simulink model "Modelo_Lazo_Cerrado_Discretizado"  (R2026b)
settings: Solver=VariableStepAuto
values from neighbouring files (symbols this model uses):
  alpha_Cu = 3.9e-3    (= 0.0039)    [coeficientes.m]
  b_eq = b_m + b_l/(r^2)    (= 2.19444444444e-05)    [coeficientes.m]
  C_ts = 0.818    [coeficientes.m]
  g = 9.80665    [coeficientes.m]
  init_I0 = 0    [coeficientes.m]
  init_Id = 0    [coeficientes.m]
  init_Iq = 0    [coeficientes.m]
  init_theta = 0    [coeficientes.m]
  init_Ts = 20    [coeficientes.m]
  init_w = 0    [coeficientes.m]
  J_eq = J_m + J_l/(r^2)    (= 4.58263888889e-05)    [coeficientes.m]
  K_et = 2*p_obs    (= 6400)    [coeficientes.m]
  K_ew = p_obs^2    (= 10240000)    [coeficientes.m]
  k_l = k_l_min + m_l*l_l    (= 1)    [coeficientes.m]
  Kd_mov = wn_mov * (2*zeta_mov + 1) * J_eq    (= 0.0916527777778)    [coeficientes.m]
  Ki_mov = wn_mov^3 * J_eq    (= 23463.1111111)    [coeficientes.m]
  Kp_mov = wn_mov^2 * (2*zeta_mov + 1) * J_eq    (= 73.3222222222)    [coeficientes.m]
  L_d = 6.6e-3    (= 0.0066)    [coeficientes.m]
  L_ls = 0.8e-3    (= 0.0008)    [coeficientes.m]
  L_q = 5.8e-3    (= 0.0058)    [coeficientes.m]
  lambda = 0.016    [coeficientes.m]
  Pp = 3    [coeficientes.m]
  r = 120.0    (= 120)    [coeficientes.m]
  R0 = abs(p)*L_ls    [coeficientes.m]
  R_sREF = 1.02    [coeficientes.m]
  R_tsamb = 146.7    [coeficientes.m]
  Rd = abs(p)*L_d    [coeficientes.m]
  Rq = abs(p)*L_q    [coeficientes.m]
  sat_V = sqrt(2/3)*V_slMAX    [coeficientes.m]
  T_sREF = 20    [coeficientes.m]
  Ts = 1e-5    (= 1e-05)    [coeficientes.m]
libraries: eeTransforms x4, eeGeneralControl x3
settings Model: Creator=fedeb  LastModifiedBy=fedeb

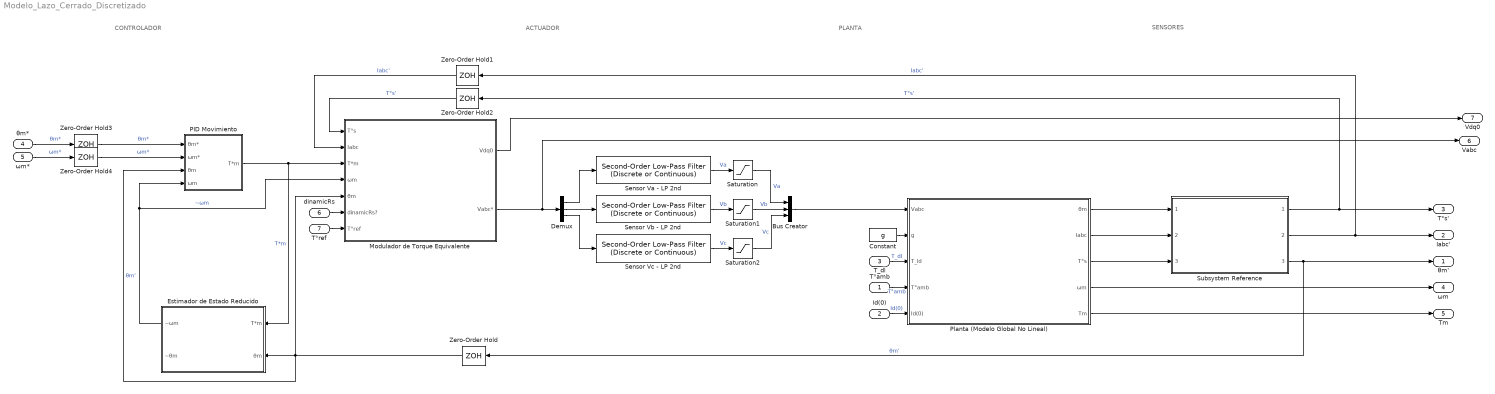
== system Modelo_Lazo_Cerrado_Discretizado ==
  note: PLANTA
  note: SENSORES
  note: CONTROLADOR
  note: ACTUADOR
  T°amb : Inport
  Id(0) : Inport  Port=2
  T_dl : Inport  Port=3
  θm* : Inport  Port=4
  ωm* : Inport  Port=5
  dinamicRs : Inport  Port=6
  T°ref : Inport  Port=7
  Bus Creator : BusCreator  Inputs=3
  Constant : Constant  Value=g
  Demux : Demux  Outputs=3
  Estimador de Estado Reducido : Subsystem
  Modulador de Torque Equivalente : Subsystem
      settings: PortSchema="{\"entries\":[{\"content\":{\"sides\":[{\"content\":{\"connectorIds\":[\"In1\",\"In3\",\"In5\",\"In2\",\"In4\",\"In6\",\"In7\"]},\"type\":\"ConnectorPlacement.EquallySpacedRectSide\",\"uuid\":\"ea9ad4ab-f607-4d37-9442-85f6cfda2486\"},{\"content\":{\"connectorIds\":[\"Out2\",\"Out1\"],\"side\":\"RIGHT\"},\"type\":\"ConnectorPlacement.EquallySpacedRectSide\",\"uuid\":\"696b5fe5-1f6c-4fc9-932e-86b56d49996f\"},{\"content\":{\"side\":\"TOP\"},\"type\":\"ConnectorPlacement.EquallySpacedRectSide\",\"uuid\":\"45e3ac4c-5a2f-4a79-9454-e497b07295c7\"}]},\"type\":\"ConnectorPlacement.EquallySpacedConnector\",\"uuid\":\"ad401c21-3c60-4ab4-96eb-f449fc93609a\"}],\"packageUris\":[\"http://schema.mathworks.com/mf0/Connector/R2020b\"],\"version\":\"1.0\"}"
  PID Movimiento : Subsystem
      settings: PortSchema="{\"entries\":[{\"content\":{\"sides\":[{\"content\":{\"connectorIds\":[\"In3\",\"In4\",\"In2\",\"In1\"]},\"type\":\"ConnectorPlacement.EquallySpacedRectSide\",\"uuid\":\"99b9ec4b-f651-40ed-8a16-085c2c4ac88d\"},{\"content\":{\"connectorIds\":[\"Out1\"],\"side\":\"RIGHT\"},\"type\":\"ConnectorPlacement.EquallySpacedRectSide\",\"uuid\":\"009a9369-fd86-4ac2-a423-7c7f1491457b\"},{\"content\":{\"side\":\"TOP\"},\"type\":\"ConnectorPlacement.EquallySpacedRectSide\",\"uuid\":\"0bc889a5-9100-482e-a11a-4c36993d76f7\"}]},\"type\":\"ConnectorPlacement.EquallySpacedConnector\",\"uuid\":\"de270b8a-8a15-46e7-87f3-10db7988a399\"}],\"packageUris\":[\"http://schema.mathworks.com/mf0/Connector/R2020b\"],\"version\":\"1.0\"}"
  Planta (Modelo Global No Lineal) : Subsystem
      settings: PortSchema="{\"entries\":[{\"content\":{\"sides\":[{\"content\":{\"connectorIds\":[\"In1\",\"In3\",\"In2\",\"In4\",\"In5\"]},\"type\":\"ConnectorPlacement.EquallySpacedRectSide\",\"uuid\":\"3481abf0-b0cb-49f6-b93f-5a31fbfa4119\"},{\"content\":{\"connectorIds\":[\"Out1\",\"Out2\",\"Out3\",\"Out4\",\"Out5\"],\"side\":\"RIGHT\"},\"type\":\"ConnectorPlacement.EquallySpacedRectSide\",\"uuid\":\"81dbc61e-d5f3-4edc-bc73-ec3d6160a008\"},{\"content\":{\"side\":\"TOP\"},\"type\":\"ConnectorPlacement.EquallySpacedRectSide\",\"uuid\":\"48e37594-92fb-4835-b4aa-9211b8b6a309\"}]},\"type\":\"ConnectorPlacement.EquallySpacedConnector\",\"uuid\":\"6c32b8e1-5803-41f4-af4e-ba3a494349ba\"}],\"packageUris\":[\"http://schema.mathworks.com/mf0/Connector/R2020b\"],\"version\":\"1.0\"}"
  Saturation : Saturate  UpperLimit=sat_V  LowerLimit=-sat_V
  Saturation1 : Saturate  UpperLimit=sat_V  LowerLimit=-sat_V
  Saturation2 : Saturate  UpperLimit=sat_V  LowerLimit=-sat_V
  Sensor Va - LP 2nd : eeGeneralControl/Second-Order Low-Pass Filter (Discrete or Continuous)  A1=A1_V  A2=A2_V  init_option=Inherited from block input  x0=0  Ts=0
      settings: LibrarySourceBlock=|
      | ee_sl_lib/General Control/Second-Order
      | Low-Pass Filter
      | (Discrete or Continuous)
  Sensor Vb - LP 2nd : eeGeneralControl/Second-Order Low-Pass Filter (Discrete or Continuous)  A1=A1_V  A2=A2_V  init_option=Inherited from block input  x0=0  Ts=0
      settings: LibrarySourceBlock=|
      | ee_sl_lib/General Control/Second-Order
      | Low-Pass Filter
      | (Discrete or Continuous)
  Sensor Vc - LP 2nd : eeGeneralControl/Second-Order Low-Pass Filter (Discrete or Continuous)  A1=A1_V  A2=A2_V  init_option=Inherited from block input  x0=0  Ts=0
      settings: LibrarySourceBlock=|
      | ee_sl_lib/General Control/Second-Order
      | Low-Pass Filter
      | (Discrete or Continuous)
  Subsystem Reference : Subsystem  ReferencedSubsystem=Sensores_Reales
  Zero-Order Hold{,1..4} (5 alike) : ZeroOrderHold  SampleTime=Ts
  θm' : Outport
  Iabc' : Outport  Port=2  OutDataTypeStr=Bus: Iabc
  T°s' : Outport  Port=3
  ωm : Outport  Port=4
  Tm : Outport  Port=5
  Vabc : Outport  Port=6  OutDataTypeStr=Bus: Vabc
  Vdq0 : Outport  Port=7  OutDataTypeStr=Bus: Vdq0
  wires:
  ωm*/1 -> Zero-Order Hold4/1  "ωm*"
  dinamicRs/1 -> Modulador de Torque Equivalente/6(dinamicRs?)
  Modulador de Torque Equivalente/2(Vdq0) -> Vdq0/1
  Planta (Modelo Global No Lineal)/5(Tm) -> Tm/1
  θm*/1 -> Zero-Order Hold3/1  "θm*"
  T_dl/1 -> Planta (Modelo Global No Lineal)/2(T_ld)  "T_dl"
  Planta (Modelo Global No Lineal)/4(ωm) -> ωm/1
  T°ref/1 -> Modulador de Torque Equivalente/7(T°ref)
  Id(0)/1 -> Planta (Modelo Global No Lineal)/5(Id(0))  "Id(0)"
  T°amb/1 -> Planta (Modelo Global No Lineal)/4(T°amb)  "T°amb"
  Subsystem Reference/2 -> Iabc'/1, Zero-Order Hold1/1  "Iabc'"
  Constant/1 -> Planta (Modelo Global No Lineal)/3(g)
  Subsystem Reference/1 -> T°s'/1, Zero-Order Hold2/1  "T°s'"
  Estimador de Estado Reducido/1(~ωm) -> Modulador de Torque Equivalente/2(ωm), PID Movimiento/1(ωm)  "~ωm"
  PID Movimiento/1(T*m) -> Modulador de Torque Equivalente/5(T*m), Estimador de Estado Reducido/1(T*m)  "T*m"
  Planta (Modelo Global No Lineal)/2(Iabc) -> Subsystem Reference/2
  Planta (Modelo Global No Lineal)/3(T°s) -> Subsystem Reference/3
  Planta (Modelo Global No Lineal)/1(θm) -> Subsystem Reference/1
  Subsystem Reference/3 -> θm'/1, Zero-Order Hold/1  "θm'"
  Sensor Va - LP 2nd/1 -> Saturation/1  "Va"
  Bus Creator/1 -> Planta (Modelo Global No Lineal)/1(Vabc)
  Saturation/1 -> Bus Creator/1  "Va"
  Sensor Vb - LP 2nd/1 -> Saturation1/1  "Vb"
  Saturation2/1 -> Bus Creator/3  "Vc"
  Demux/3 -> Sensor Vc - LP 2nd/1
  Modulador de Torque Equivalente/1(Vabc*) -> Demux/1, Vabc/1
  Demux/2 -> Sensor Vb - LP 2nd/1
  Demux/1 -> Sensor Va - LP 2nd/1
  Sensor Vc - LP 2nd/1 -> Saturation2/1  "Vc"
  Saturation1/1 -> Bus Creator/2  "Vb"
  Zero-Order Hold/1 -> Estimador de Estado Reducido/2(θm), PID Movimiento/2(θm), Modulador de Torque Equivalente/4(θm)  "θm'"
  Zero-Order Hold1/1 -> Modulador de Torque Equivalente/3(Iabc)  "Iabc'"
  Zero-Order Hold2/1 -> Modulador de Torque Equivalente/1(T°s)  "T°s'"
  Zero-Order Hold3/1 -> PID Movimiento/3(θm*)  "θm*"
  Zero-Order Hold4/1 -> PID Movimiento/4(ωm*)  "ωm*"

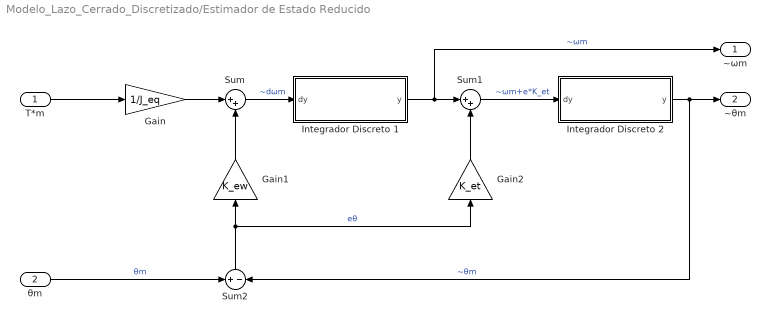
== system Modelo_Lazo_Cerrado_Discretizado/Estimador de Estado Reducido ==
  T*m : Inport
  θm : Inport  Port=2
  Gain : Gain  Gain=1/J_eq
  Gain1 : Gain  Gain=K_ew
  Gain2 : Gain  Gain=K_et
  Integrador Discreto 1 : Subsystem
  Integrador Discreto 2 : Subsystem
  Sum : Sum  Inputs=|++
  Sum1 : Sum  Inputs=|++
  Sum2 : Sum  Inputs=+-
  ~ωm : Outport
  ~θm : Outport  Port=2
  wires:
  T*m/1 -> Gain/1
  Gain/1 -> Sum/1
  Sum/1 -> Integrador Discreto 1/1(dy)  "~dωm"
  Sum1/1 -> Integrador Discreto 2/1(dy)  "~ωm+e*K_et"
  Integrador Discreto 1/1(y) -> ~ωm/1, Sum1/1  "~ωm"
  Gain1/1 -> Sum/2
  Gain2/1 -> Sum1/2
  Sum2/1 -> Gain1/1, Gain2/1  "eθ"
  θm/1 -> Sum2/1  "θm"
  Integrador Discreto 2/1(y) -> Sum2/2, ~θm/1  "~θm"

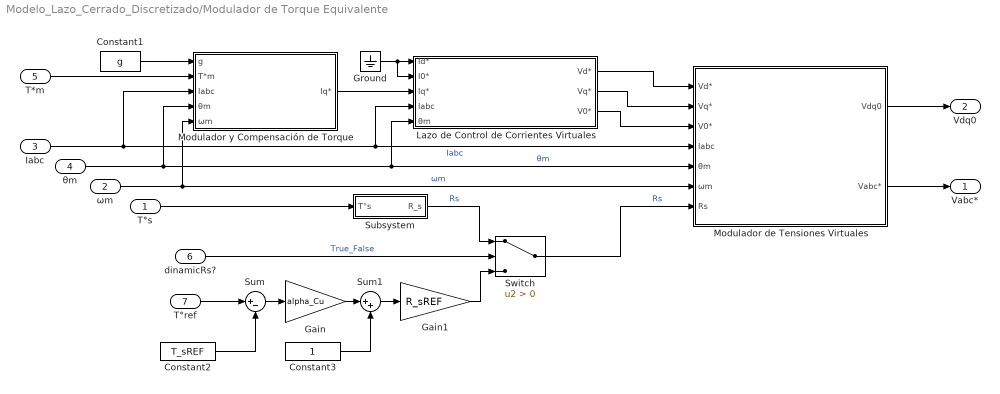
== system Modelo_Lazo_Cerrado_Discretizado/Modulador de Torque Equivalente ==
  T°s : Inport
  ωm : Inport  Port=2
  Iabc : Inport  Port=3
  θm : Inport  Port=4
  T*m : Inport  Port=5
  dinamicRs? : Inport  Port=6
  T°ref : Inport  Port=7
  Constant1 : Constant  Value=g
  Constant2 : Constant  Value=T_sREF
  Constant3 : Constant
  Gain : Gain  Gain=alpha_Cu
  Gain1 : Gain  Gain=R_sREF
  Ground : Ground
  Lazo de Control de Corrientes Virtuales : Subsystem
      settings: PortSchema="{\"entries\":[{\"content\":{\"sides\":[{\"content\":{\"connectorIds\":[\"In2\",\"In3\",\"In1\",\"In4\",\"In5\"]},\"type\":\"ConnectorPlacement.EquallySpacedRectSide\",\"uuid\":\"7378df2b-1b9c-42cd-9ef6-9bfa4de31228\"},{\"content\":{\"connectorIds\":[\"Out2\",\"Out1\",\"Out3\"],\"side\":\"RIGHT\"},\"type\":\"ConnectorPlacement.EquallySpacedRectSide\",\"uuid\":\"75ac4e09-b611-4ee2-aa1e-16791f3f98b8\"},{\"content\":{\"side\":\"TOP\"},\"type\":\"ConnectorPlacement.EquallySpacedRectSide\",\"uuid\":\"c32b7829-5b6a-417b-8aae-eaa4caf59bef\"}]},\"type\":\"ConnectorPlacement.EquallySpacedConnector\",\"uuid\":\"1d84f5ff-db01-492a-bfe1-22065b3eebb0\"}],\"packageUris\":[\"http://schema.mathworks.com/mf0/Connector/R2020b\"],\"version\":\"1.0\"}"
  Modulador de Tensiones Virtuales : Subsystem
      settings: PortSchema="{\"entries\":[{\"content\":{\"sides\":[{\"content\":{\"connectorIds\":[\"In2\",\"In1\",\"In3\",\"In6\",\"In7\",\"In5\",\"In4\"]},\"type\":\"ConnectorPlacement.EquallySpacedRectSide\",\"uuid\":\"561a625a-719f-47d4-85d3-a88e423068dd\"},{\"content\":{\"connectorIds\":[\"Out2\",\"Out1\"],\"side\":\"RIGHT\"},\"type\":\"ConnectorPlacement.EquallySpacedRectSide\",\"uuid\":\"c1cdd74a-6c1d-470e-a6ac-8d72e83b5cc5\"},{\"content\":{\"side\":\"TOP\"},\"type\":\"ConnectorPlacement.EquallySpacedRectSide\",\"uuid\":\"c5935c6f-534c-46b9-aa64-6d6dabbbb210\"}]},\"type\":\"ConnectorPlacement.EquallySpacedConnector\",\"uuid\":\"b0debde9-6e18-4e06-b0c4-28c9c51e472d\"}],\"packageUris\":[\"http://schema.mathworks.com/mf0/Connector/R2020b\"],\"version\":\"1.0\"}"
  Modulador y Compensación de Torque : Subsystem
      settings: PortSchema="{\"entries\":[{\"content\":{\"sides\":[{\"content\":{\"connectorIds\":[\"In5\",\"In1\",\"In2\",\"In3\",\"In4\"]},\"type\":\"ConnectorPlacement.EquallySpacedRectSide\",\"uuid\":\"ea9ad4ab-f607-4d37-9442-85f6cfda2486\"},{\"content\":{\"connectorIds\":[\"Out1\"],\"side\":\"RIGHT\"},\"type\":\"ConnectorPlacement.EquallySpacedRectSide\",\"uuid\":\"696b5fe5-1f6c-4fc9-932e-86b56d49996f\"},{\"content\":{\"side\":\"TOP\"},\"type\":\"ConnectorPlacement.EquallySpacedRectSide\",\"uuid\":\"45e3ac4c-5a2f-4a79-9454-e497b07295c7\"}]},\"type\":\"ConnectorPlacement.EquallySpacedConnector\",\"uuid\":\"ad401c21-3c60-4ab4-96eb-f449fc93609a\"}],\"packageUris\":[\"http://schema.mathworks.com/mf0/Connector/R2020b\"],\"version\":\"1.0\"}"
  Subsystem : Subsystem
  Sum : Sum  Inputs=|+-
  Sum1 : Sum  Inputs=|++
  Switch : Switch  Criteria=u2 > Threshold  SaturateOnIntegerOverflow=off  InputSameDT=off
  Vabc* : Outport
  Vdq0 : Outport  Port=2
  wires:
  Lazo de Control de Corrientes Virtuales/1(Vq*) -> Modulador de Tensiones Virtuales/1(Vq*)
  Lazo de Control de Corrientes Virtuales/2(Vd*) -> Modulador de Tensiones Virtuales/2(Vd*)
  Lazo de Control de Corrientes Virtuales/3(V0*) -> Modulador de Tensiones Virtuales/3(V0*)
  Modulador y Compensación de Torque/1(Iq*) -> Lazo de Control de Corrientes Virtuales/1(Iq*)
  T*m/1 -> Modulador y Compensación de Torque/1(T*m)
  θm/1 -> Modulador de Tensiones Virtuales/7(θm), Lazo de Control de Corrientes Virtuales/5(θm), Modulador y Compensación de Torque/3(θm)  "θm"
  ωm/1 -> Modulador de Tensiones Virtuales/5(ωm), Modulador y Compensación de Torque/4(ωm)  "ωm"
  Modulador de Tensiones Virtuales/1(Vabc*) -> Vabc*/1
  Ground/1 -> Lazo de Control de Corrientes Virtuales/2(Id*), Lazo de Control de Corrientes Virtuales/3(I0*)
  Iabc/1 -> Modulador de Tensiones Virtuales/6(Iabc), Lazo de Control de Corrientes Virtuales/4(Iabc), Modulador y Compensación de Torque/2(Iabc)  "Iabc"
  T°s/1 -> Subsystem/1(T°s)
  Subsystem/1(R_s) -> Switch/1  "Rs"
  dinamicRs?/1 -> Switch/2  "True_False"
  Switch/1 -> Modulador de Tensiones Virtuales/4(Rs)  "Rs"
  Gain1/1 -> Switch/3
  Modulador de Tensiones Virtuales/2(Vdq0) -> Vdq0/1
  Constant1/1 -> Modulador y Compensación de Torque/5(g)
  T°ref/1 -> Sum/1
  Constant2/1 -> Sum/2
  Sum/1 -> Gain/1
  Gain/1 -> Sum1/1
  Constant3/1 -> Sum1/2
  Sum1/1 -> Gain1/1

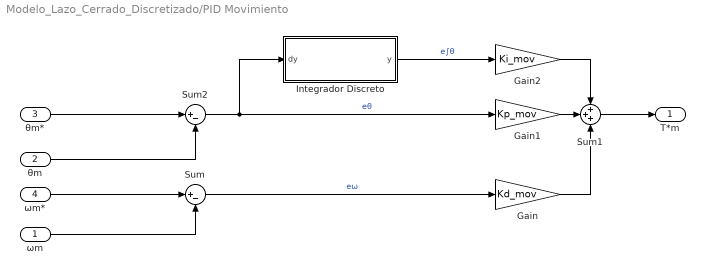
== system Modelo_Lazo_Cerrado_Discretizado/PID Movimiento ==
  ωm : Inport  Unit=rad/s
  θm : Inport  Port=2
  θm* : Inport  Port=3  Unit=rad/s
  ωm* : Inport  Port=4  Unit=rad/s
  Gain : Gain  Gain=Kd_mov
  Gain1 : Gain  Gain=Kp_mov
  Gain2 : Gain  Gain=Ki_mov
  Integrador Discreto : Subsystem
  Sum : Sum  Inputs=|+-
  Sum1 : Sum  Inputs=+++
  Sum2 : Sum  Inputs=|+-
  T*m : Outport
  wires:
  Gain1/1 -> Sum1/2
  Sum1/1 -> T*m/1
  Gain2/1 -> Sum1/1
  Gain/1 -> Sum1/3
  θm*/1 -> Sum2/1
  Sum/1 -> Gain/1  "eω"
  θm/1 -> Sum2/2
  ωm*/1 -> Sum/1
  ωm/1 -> Sum/2
  Integrador Discreto/1(y) -> Gain2/1  "e∫θ"
  Sum2/1 -> Integrador Discreto/1(dy), Gain1/1  "eθ"

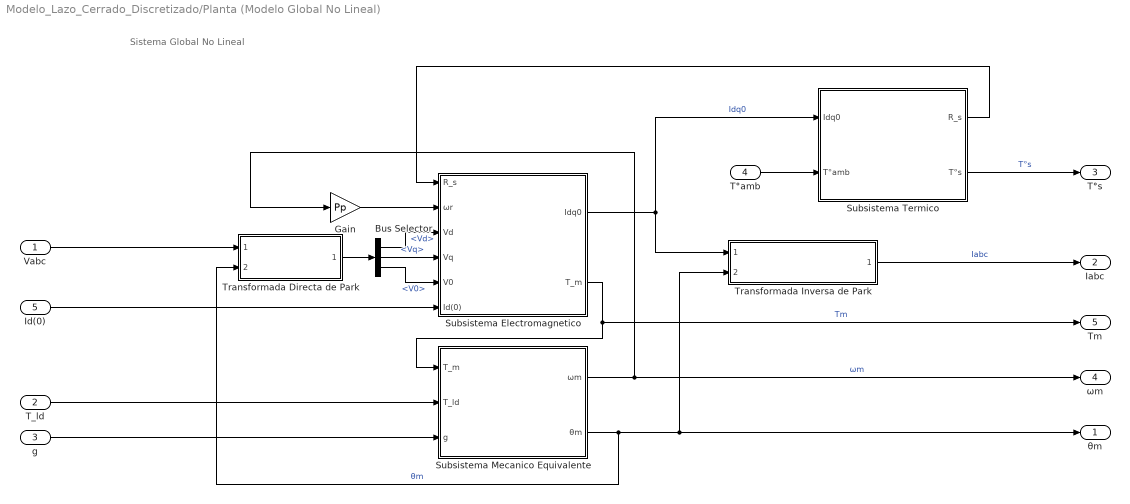
== system Modelo_Lazo_Cerrado_Discretizado/Planta (Modelo Global No Lineal) ==
  note: Sistema Global No Lineal
  Vabc : Inport  OutDataTypeStr=Bus: Vabc
  T_ld : Inport  Port=2
  g : Inport  Port=3
  T°amb : Inport  Port=4
  Id(0) : Inport  Port=5
  Bus Selector : BusSelector  OutputSignals=Vd,Vq,V0
  Gain : Gain  Gain=Pp
  Subsistema Electromagnetico : Subsystem
  Subsistema Mecanico Equivalente : Subsystem
  Subsistema Termico : Subsystem
  Transformada Directa de Park : Subsystem  ReferencedSubsystem=Transformada_Directa_de_Park_V
  Transformada Inversa de Park : Subsystem  ReferencedSubsystem=Transformada_Inversa_de_Park_I
  θm : Outport
  Iabc : Outport  Port=2  OutDataTypeStr=Bus: Iabc
  T°s : Outport  Port=3
  ωm : Outport  Port=4
  Tm : Outport  Port=5
  wires:
  Subsistema Termico/2(T°s) -> T°s/1  "T°s"
  Subsistema Electromagnetico/1(Idq0) -> Subsistema Termico/1(Idq0), Transformada Inversa de Park/1  "Idq0"
  Subsistema Mecanico Equivalente/1(ωm) -> Gain/1, ωm/1  "ωm"
  Subsistema Mecanico Equivalente/2(θm) -> Transformada Directa de Park/2, Transformada Inversa de Park/2, θm/1  "θm"
  Subsistema Electromagnetico/2(T_m) -> Subsistema Mecanico Equivalente/1(T_m), Tm/1  "Tm"
  Subsistema Termico/1(R_s) -> Subsistema Electromagnetico/1(R_s)
  Gain/1 -> Subsistema Electromagnetico/2(ωr)
  T_ld/1 -> Subsistema Mecanico Equivalente/2(T_ld)
  Vabc/1 -> Transformada Directa de Park/1
  T°amb/1 -> Subsistema Termico/2(T°amb)
  g/1 -> Subsistema Mecanico Equivalente/3(g)
  Transformada Directa de Park/1 -> Bus Selector/1
  Bus Selector/1 -> Subsistema Electromagnetico/3(Vd)  "<Vd>"
  Bus Selector/2 -> Subsistema Electromagnetico/4(Vq)  "<Vq>"
  Bus Selector/3 -> Subsistema Electromagnetico/5(V0)  "<V0>"
  Transformada Inversa de Park/1 -> Iabc/1  "Iabc"
  Id(0)/1 -> Subsistema Electromagnetico/6(Id(0))

== system Modelo_Lazo_Cerrado_Discretizado/Estimador de Estado Reducido/Integrador Discreto 1 ==
  dy : Inport
  Gain : Gain  Gain=Ts/2
  Sum : Sum  Inputs=|++
  Sum1 : Sum  Inputs=|++
  Unit Delay : UnitDelay  SampleTime=Ts
  Unit Delay1 : UnitDelay  SampleTime=Ts
  y : Outport
  wires:
  dy/1 -> Unit Delay/1, Sum/1
  Unit Delay/1 -> Sum/2
  Sum/1 -> Gain/1
  Gain/1 -> Sum1/1
  Sum1/1 -> y/1, Unit Delay1/1
  Unit Delay1/1 -> Sum1/2

== system Modelo_Lazo_Cerrado_Discretizado/Estimador de Estado Reducido/Integrador Discreto 2 ==
  dy : Inport
  Gain : Gain  Gain=Ts/2
  Sum : Sum  Inputs=|++
  Sum1 : Sum  Inputs=|++
  Unit Delay : UnitDelay  SampleTime=Ts
  Unit Delay1 : UnitDelay  SampleTime=Ts
  y : Outport
  wires:
  Unit Delay1/1 -> Sum1/2
  Sum1/1 -> Unit Delay1/1, y/1
  Gain/1 -> Sum1/1
  Sum/1 -> Gain/1
  Unit Delay/1 -> Sum/2
  dy/1 -> Sum/1, Unit Delay/1

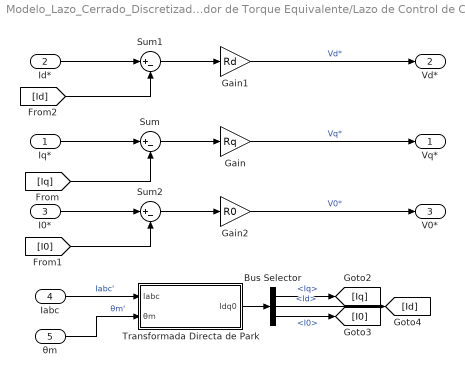
== system Modelo_Lazo_Cerrado_Discretizado/Modulador de Torque Equivalente/Lazo de Control de Corrientes Virtuales ==
  Iq* : Inport
  Id* : Inport  Port=2
  I0* : Inport  Port=3
  Iabc : Inport  Port=4
  θm : Inport  Port=5
  Bus Selector : BusSelector  OutputSignals=Iq,Id,I0
  Gain : Gain  Gain=Rq
  Gain1 : Gain  Gain=Rd
  Gain2 : Gain  Gain=R0
  Sum : Sum  Inputs=|+-
  Sum1 : Sum  Inputs=|+-
  Sum2 : Sum  Inputs=|+-
  Transformada Directa de Park : Subsystem
  Vq* : Outport
  Vd* : Outport  Port=2
  V0* : Outport  Port=3
  wires:
  Bus Selector/1 -> [Iq]  "<Iq>"
  θm/1 -> Transformada Directa de Park/2(θm)  "θm'"
  Iabc/1 -> Transformada Directa de Park/1(Iabc)  "Iabc'"
  Transformada Directa de Park/1(Idq0) -> Bus Selector/1
  Bus Selector/3 -> [I0]  "<I0>"
  Bus Selector/2 -> [Id]  "<Id>"
  I0*/1 -> Sum2/1
  [I0] -> Sum2/2
  Sum2/1 -> Gain2/1
  Gain2/1 -> V0*/1  "V0*"
  Sum/1 -> Gain/1
  [Id] -> Sum1/2
  [Iq] -> Sum/2
  Gain1/1 -> Vd*/1  "Vd*"
  Iq*/1 -> Sum/1
  Id*/1 -> Sum1/1
  Gain/1 -> Vq*/1  "Vq*"
  Sum1/1 -> Gain1/1

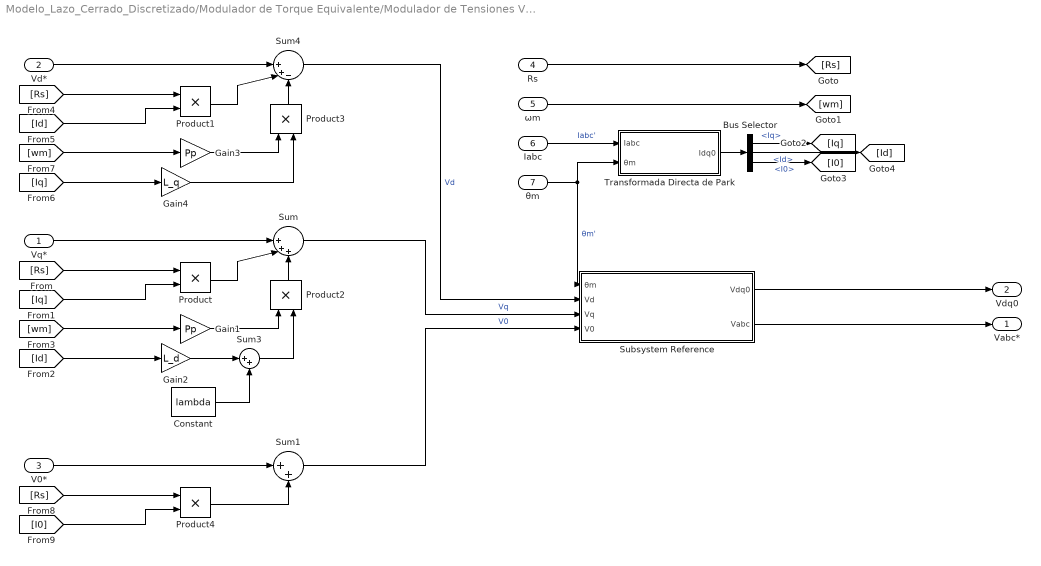
== system Modelo_Lazo_Cerrado_Discretizado/Modulador de Torque Equivalente/Modulador de Tensiones Virtuales ==
  Vq* : Inport
  Vd* : Inport  Port=2
  V0* : Inport  Port=3
  Rs : Inport  Port=4
  ωm : Inport  Port=5
  Iabc : Inport  Port=6
  θm : Inport  Port=7
  Bus Selector : BusSelector  OutputSignals=Iq,Id,I0
  Constant : Constant  Value=lambda
  Gain1 : Gain  Gain=Pp
  Gain2 : Gain  Gain=L_d
  Gain3 : Gain  Gain=Pp
  Gain4 : Gain  Gain=L_q
  Product{,1..4} (5 alike) : Product
  Subsystem Reference : Subsystem
  Sum : Sum  Inputs=||+++
  Sum1 : Sum  Inputs=|++
  Sum3 : Sum  Inputs=|++
  Sum4 : Sum  Inputs=||++-
  Transformada Directa de Park : Subsystem
  Vabc* : Outport
  Vdq0 : Outport  Port=2
  wires:
  Product4/1 -> Sum1/2
  V0*/1 -> Sum1/1
  [Rs] -> Product4/1
  [I0] -> Product4/2
  [Id] -> Product1/2
  Product3/1 -> Sum4/3
  Gain4/1 -> Product3/2
  Vd*/1 -> Sum4/1
  [Rs] -> Product1/1
  Gain3/1 -> Product3/1
  [Iq] -> Gain4/1
  Product1/1 -> Sum4/2
  [wm] -> Gain3/1
  [Iq] -> Product/2
  Gain1/1 -> Product2/1
  Sum3/1 -> Product2/2
  [wm] -> Gain1/1
  Product2/1 -> Sum/3
  Gain2/1 -> Sum3/1
  [Id] -> Gain2/1
  Constant/1 -> Sum3/2
  Product/1 -> Sum/2
  [Rs] -> Product/1
  Vq*/1 -> Sum/1
  Bus Selector/2 -> [Id]  "<Id>"
  Bus Selector/3 -> [I0]  "<I0>"
  Bus Selector/1 -> [Iq]  "<Iq>"
  ωm/1 -> [wm]
  Rs/1 -> [Rs]
  Subsystem Reference/2(Vabc) -> Vabc*/1
  θm/1 -> Subsystem Reference/1(θm), Transformada Directa de Park/2(θm)  "θm'"
  Transformada Directa de Park/1(Idq0) -> Bus Selector/1
  Iabc/1 -> Transformada Directa de Park/1(Iabc)  "Iabc'"
  Subsystem Reference/1(Vdq0) -> Vdq0/1
  Sum4/1 -> Subsystem Reference/2(Vd)  "Vd"
  Sum/1 -> Subsystem Reference/3(Vq)  "Vq"
  Sum1/1 -> Subsystem Reference/4(V0)  "V0"

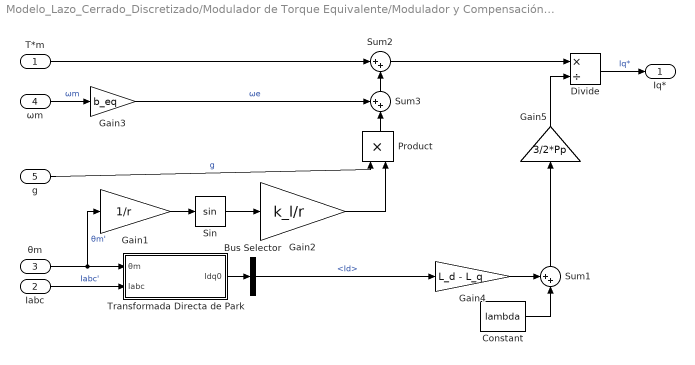
== system Modelo_Lazo_Cerrado_Discretizado/Modulador de Torque Equivalente/Modulador y Compensación de Torque ==
  T*m : Inport
  Iabc : Inport  Port=2
  θm : Inport  Port=3
  ωm : Inport  Port=4
  g : Inport  Port=5
  Bus Selector : BusSelector  OutputSignals=Id
  Constant : Constant  Value=lambda
  Divide : Product  Inputs=*/
  Gain1 : Gain  Gain=1/r
  Gain2 : Gain  Gain=k_l/r
  Gain3 : Gain  Gain=b_eq
  Gain4 : Gain  Gain=L_d - L_q
  Gain5 : Gain  Gain=3/2*Pp
  Product : Product
  Sin : Trigonometry
  Sum1 : Sum  Inputs=++|
  Sum2 : Sum  Inputs=|++
  Sum3 : Sum  Inputs=++|
  Transformada Directa de Park : Subsystem
  Iq* : Outport
  wires:
  Divide/1 -> Iq*/1  "Iq*"
  T*m/1 -> Sum2/1
  Iabc/1 -> Transformada Directa de Park/2(Iabc)  "Iabc'"
  θm/1 -> Gain1/1, Transformada Directa de Park/1(θm)  "θm'"
  Transformada Directa de Park/1(Idq0) -> Bus Selector/1
  Gain4/1 -> Sum1/1
  Constant/1 -> Sum1/2
  Sum1/1 -> Gain5/1
  Sum2/1 -> Divide/1
  Gain5/1 -> Divide/2
  Bus Selector/1 -> Gain4/1  "<Id>"
  Gain1/1 -> Sin/1
  Sin/1 -> Gain2/1
  Product/1 -> Sum3/2
  Gain2/1 -> Product/2
  g/1 -> Product/1  "g"
  ωm/1 -> Gain3/1  "ωm"
  Gain3/1 -> Sum3/1  "ωe"
  Sum3/1 -> Sum2/2

== system Modelo_Lazo_Cerrado_Discretizado/Modulador de Torque Equivalente/Subsystem ==
  T°s : Inport
  Constant1 : Constant  Value=T_sREF
  Constant2 : Constant
  Gain5 : Gain  Gain=alpha_Cu
  Gain6 : Gain  Gain=R_sREF
  Sum3 : Sum  Inputs=+-|
  Sum4 : Sum  Inputs=|++
  R_s : Outport
  wires:
  T°s/1 -> Sum3/1
  Gain5/1 -> Sum4/1
  Gain6/1 -> R_s/1  "R_s"
  Constant1/1 -> Sum3/2
  Constant2/1 -> Sum4/2
  Sum4/1 -> Gain6/1
  Sum3/1 -> Gain5/1

== system Modelo_Lazo_Cerrado_Discretizado/PID Movimiento/Integrador Discreto ==
  dy : Inport
  Gain : Gain  Gain=Ts/2
  Sum : Sum  Inputs=|++
  Sum1 : Sum  Inputs=|++
  Unit Delay : UnitDelay  SampleTime=Ts
  Unit Delay1 : UnitDelay  SampleTime=Ts
  y : Outport
  wires:
  dy/1 -> Unit Delay/1, Sum/1
  Unit Delay/1 -> Sum/2
  Sum/1 -> Gain/1
  Gain/1 -> Sum1/1
  Sum1/1 -> y/1, Unit Delay1/1
  Unit Delay1/1 -> Sum1/2

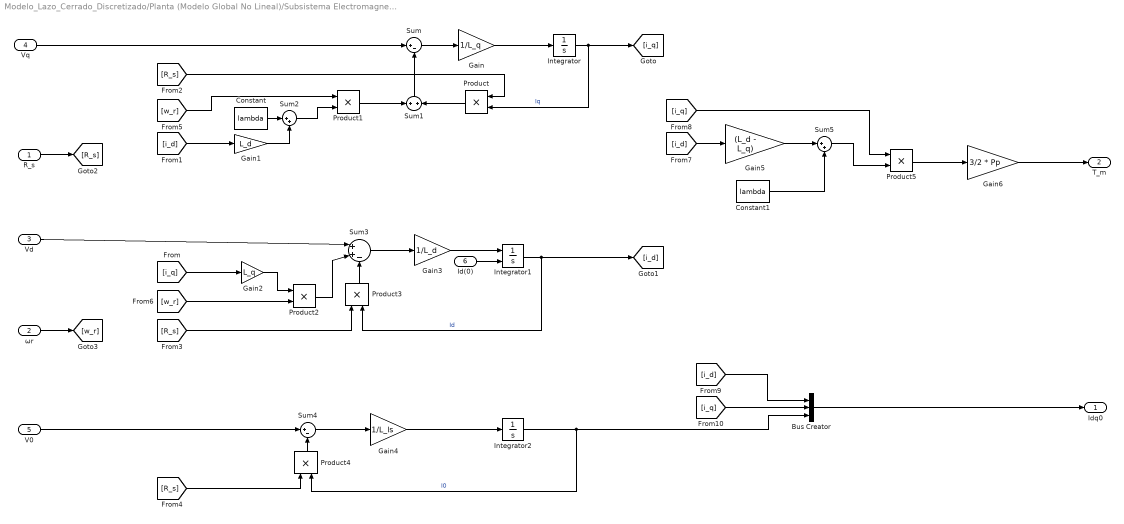
== system Modelo_Lazo_Cerrado_Discretizado/Planta (Modelo Global No Lineal)/Subsistema Electromagnetico ==
  R_s : Inport
  ωr : Inport  Port=2
  Vd : Inport  Port=3
  Vq : Inport  Port=4
  V0 : Inport  Port=5
  Id(0) : Inport  Port=6
  Bus Creator : BusCreator  Inputs=3
  Constant : Constant  Value=lambda
  Constant1 : Constant  Value=lambda
  Gain : Gain  Gain=1/L_q
  Gain1 : Gain  Gain=L_d
  Gain2 : Gain  Gain=L_q
  Gain3 : Gain  Gain=1/L_d
  Gain4 : Gain  Gain=1/L_ls
  Gain5 : Gain  Gain=(L_d - L_q)
  Gain6 : Gain  Gain=3/2 * Pp
  Integrator : Integrator  InitialCondition=init_Iq
  Integrator1 : Integrator  InitialConditionSource=external  InitialCondition=init_Id
  Integrator2 : Integrator  InitialCondition=init_I0
  Product{,1..5} (6 alike) : Product
  Sum : Sum  Inputs=|+-
  Sum1 : Sum
  Sum2 : Sum  Inputs=|++
  Sum3 : Sum  Inputs=|++-
  Sum4 : Sum  Inputs=|+-
  Sum5 : Sum  Inputs=|++
  Idq0 : Outport
  T_m : Outport  Port=2
  wires:
  [w_r] -> Product2/2
  Gain2/1 -> Product2/1
  Product2/1 -> Sum3/2
  [i_q] -> Gain2/1
  Integrator/1 -> Product/2, [i_q]  "Iq"
  [R_s] -> Product/1
  Product/1 -> Sum1/2
  Sum1/1 -> Sum/2
  Product1/1 -> Sum1/1
  Gain1/1 -> Sum2/2
  Sum2/1 -> Product1/2
  Constant/1 -> Sum2/1
  Sum/1 -> Gain/1
  Vq/1 -> Sum/1
  Gain/1 -> Integrator/1
  Product3/1 -> Sum3/3
  Gain3/1 -> Integrator1/1
  Sum3/1 -> Gain3/1
  Vd/1 -> Sum3/1
  Product4/1 -> Sum4/2
  Integrator2/1 -> Bus Creator/3, Product4/2  "I0"
  Gain4/1 -> Integrator2/1
  Sum4/1 -> Gain4/1
  V0/1 -> Sum4/1
  Gain5/1 -> Sum5/1
  Sum5/1 -> Product5/2
  Integrator1/1 -> [i_d], Product3/2  "Id"
  Constant1/1 -> Sum5/2
  Product5/1 -> Gain6/1
  Gain6/1 -> T_m/1
  [i_d] -> Gain1/1
  R_s/1 -> [R_s]
  [R_s] -> Product3/1
  [R_s] -> Product4/1
  ωr/1 -> [w_r]
  [w_r] -> Product1/1
  [i_d] -> Gain5/1
  [i_q] -> Product5/1
  Bus Creator/1 -> Idq0/1
  Id(0)/1 -> Integrator1/2
  [i_d] -> Bus Creator/1
  [i_q] -> Bus Creator/2

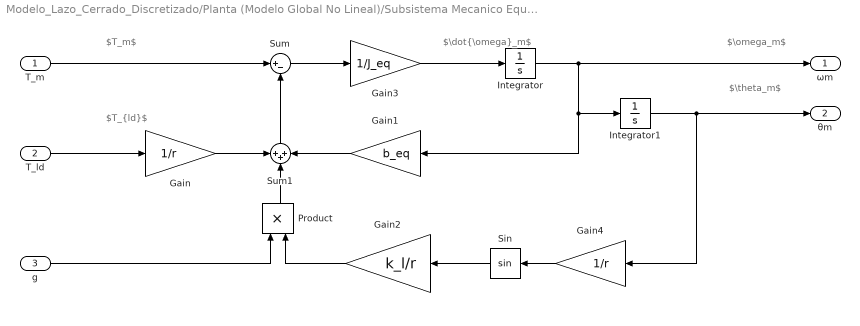
== system Modelo_Lazo_Cerrado_Discretizado/Planta (Modelo Global No Lineal)/Subsistema Mecanico Equivalente ==
  note: $T_m$
  note: $T_{ld}$
  note: $\dot{\omega}_m$
  note: $\omega_m$
  note: $\theta_m$
  T_m : Inport
  T_ld : Inport  Port=2
  g : Inport  Port=3
  Gain : Gain  Gain=1/r
  Gain1 : Gain  Gain=b_eq
  Gain2 : Gain  Gain=k_l/r
  Gain3 : Gain  Gain=1/J_eq
  Gain4 : Gain  Gain=1/r
  Integrator : Integrator  InitialCondition=init_w
  Integrator1 : Integrator  InitialCondition=init_theta
  Product : Product
  Sin : Trigonometry
  Sum : Sum  Inputs=|+-
  Sum1 : Sum  Inputs=+++
  ωm : Outport
  θm : Outport  Port=2
  wires:
  Sum/1 -> Gain3/1
  T_m/1 -> Sum/1
  Sum1/1 -> Sum/2
  Gain2/1 -> Product/2
  Gain/1 -> Sum1/1
  Sin/1 -> Gain2/1
  Gain1/1 -> Sum1/3
  Gain3/1 -> Integrator/1
  Gain4/1 -> Sin/1
  T_ld/1 -> Gain/1
  Product/1 -> Sum1/2
  g/1 -> Product/1
  Integrator/1 -> ωm/1, Integrator1/1, Gain1/1
  Integrator1/1 -> Gain4/1, θm/1

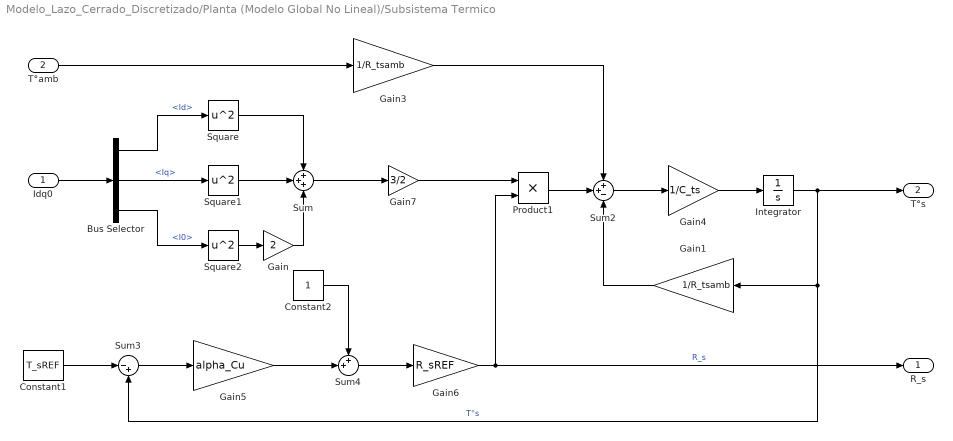
== system Modelo_Lazo_Cerrado_Discretizado/Planta (Modelo Global No Lineal)/Subsistema Termico ==
  Idq0 : Inport
  T°amb : Inport  Port=2
  Bus Selector : BusSelector  OutputSignals=Id,Iq,I0
  Constant1 : Constant  Value=T_sREF
  Constant2 : Constant
  Gain : Gain  Gain=2
  Gain1 : Gain  Gain=1/R_tsamb
  Gain3 : Gain  Gain=1/R_tsamb
  Gain4 : Gain  Gain=1/C_ts
  Gain5 : Gain  Gain=alpha_Cu
  Gain6 : Gain  Gain=R_sREF
  Gain7 : Gain  Gain=3/2
  Integrator : Integrator  InitialCondition=init_Ts
  Product1 : Product
  Square : Math  Operator=square
  Square1 : Math  Operator=square
  Square2 : Math  Operator=square
  Sum : Sum  Inputs=+++
  Sum2 : Sum  Inputs=++-
  Sum3 : Sum  Inputs=|-+
  Sum4 : Sum  Inputs=++|
  R_s : Outport
  T°s : Outport  Port=2
  wires:
  Bus Selector/2 -> Square1/1  "<Iq>"
  Square1/1 -> Sum/2
  Integrator/1 -> Sum3/2, Gain1/1, T°s/1  "T°s"
  Gain6/1 -> R_s/1, Product1/2  "R_s"
  Gain7/1 -> Product1/1
  Sum4/1 -> Gain6/1
  Constant1/1 -> Sum3/1
  Gain/1 -> Sum/3
  Gain5/1 -> Sum4/2
  Sum3/1 -> Gain5/1
  T°amb/1 -> Gain3/1
  Sum/1 -> Gain7/1
  Square2/1 -> Gain/1
  Sum2/1 -> Gain4/1
  Square/1 -> Sum/1
  Product1/1 -> Sum2/2
  Gain4/1 -> Integrator/1
  Gain1/1 -> Sum2/3
  Gain3/1 -> Sum2/1
  Idq0/1 -> Bus Selector/1
  Constant2/1 -> Sum4/1
  Bus Selector/1 -> Square/1  "<Id>"
  Bus Selector/3 -> Square2/1  "<I0>"

== system Modelo_Lazo_Cerrado_Discretizado/Modulador de Torque Equivalente/Lazo de Control de Corrientes Virtuales/Transformada Directa de Park ==
  Iabc : Inport
  θm : Inport  Port=2
  Bus Creator : BusCreator  Inputs=3
  Demux : Demux  Outputs=3
  Gain3 : Gain  Gain=Pp
  Park Transform : eeTransforms/Park Transform  AxisAlignment=Q-axis  PowerInvariant=off
      settings: LibrarySourceBlock=|
      | ee_sl_lib/Mathematical
      | Transforms/Park Transform
  Idq0 : Outport
  wires:
  θm/1 -> Gain3/1
  Iabc/1 -> Park Transform/1
  Bus Creator/1 -> Idq0/1
  Demux/2 -> Bus Creator/2  "Iq"
  Demux/3 -> Bus Creator/3  "I0"
  Demux/1 -> Bus Creator/1  "Id"
  Park Transform/1 -> Demux/1  "Idq0"
  Gain3/1 -> Park Transform/2

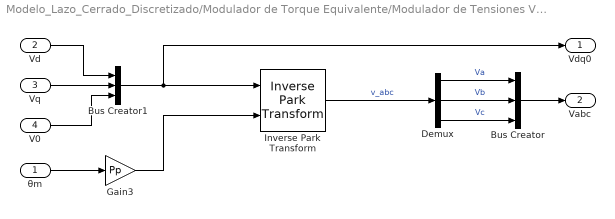
== system Modelo_Lazo_Cerrado_Discretizado/Modulador de Torque Equivalente/Modulador de Tensiones Virtuales/Subsystem Reference ==
  θm : Inport
  Vd : Inport  Port=2
  Vq : Inport  Port=3
  V0 : Inport  Port=4
  Bus Creator : BusCreator  Inputs=3
  Bus Creator1 : BusCreator  Inputs=3
  Demux : Demux  Outputs=3
  Gain3 : Gain  Gain=Pp
  Inverse Park Transform : eeTransforms/Inverse Park Transform  AxisAlignment=Q-axis  PowerInvariant=off
      settings: LibrarySourceBlock=|
      | ee_sl_lib/Mathematical
      | Transforms/Inverse
      | Park Transform
  Vdq0 : Outport
  Vabc : Outport  Port=2
  wires:
  Gain3/1 -> Inverse Park Transform/2
  Inverse Park Transform/1 -> Demux/1  "v_abc"
  Demux/1 -> Bus Creator/1  "Va"
  Demux/3 -> Bus Creator/3  "Vc"
  Demux/2 -> Bus Creator/2  "Vb"
  Bus Creator/1 -> Vabc/1
  θm/1 -> Gain3/1
  Vd/1 -> Bus Creator1/1
  Vq/1 -> Bus Creator1/2
  V0/1 -> Bus Creator1/3
  Bus Creator1/1 -> Vdq0/1, Inverse Park Transform/1

== system Modelo_Lazo_Cerrado_Discretizado/Modulador de Torque Equivalente/Modulador de Tensiones Virtuales/Transformada Directa de Park ==
  Iabc : Inport
  θm : Inport  Port=2
  Bus Creator : BusCreator  Inputs=3
  Demux : Demux  Outputs=3
  Gain3 : Gain  Gain=Pp
  Park Transform : eeTransforms/Park Transform  AxisAlignment=Q-axis  PowerInvariant=off
      settings: LibrarySourceBlock=|
      | ee_sl_lib/Mathematical
      | Transforms/Park Transform
  Idq0 : Outport
  wires:
  Gain3/1 -> Park Transform/2
  Park Transform/1 -> Demux/1  "Idq0"
  Demux/1 -> Bus Creator/1  "Id"
  Demux/3 -> Bus Creator/3  "I0"
  Demux/2 -> Bus Creator/2  "Iq"
  Bus Creator/1 -> Idq0/1
  Iabc/1 -> Park Transform/1
  θm/1 -> Gain3/1

== system Modelo_Lazo_Cerrado_Discretizado/Modulador de Torque Equivalente/Modulador y Compensación de Torque/Transformada Directa de Park ==
  θm : Inport
  Iabc : Inport  Port=2
  Bus Creator : BusCreator  Inputs=3
  Demux : Demux  Outputs=3
  Gain3 : Gain  Gain=Pp
  Park Transform : eeTransforms/Park Transform  AxisAlignment=Q-axis  PowerInvariant=off
      settings: LibrarySourceBlock=|
      | ee_sl_lib/Mathematical
      | Transforms/Park Transform
  Idq0 : Outport
  wires:
  θm/1 -> Gain3/1
  Iabc/1 -> Park Transform/1
  Bus Creator/1 -> Idq0/1
  Demux/2 -> Bus Creator/2  "Iq"
  Demux/3 -> Bus Creator/3  "I0"
  Demux/1 -> Bus Creator/1  "Id"
  Park Transform/1 -> Demux/1  "Idq0"
  Gain3/1 -> Park Transform/2
